simulink model "REF"  (R2025b)
settings: Solver=VariableStepAuto  StartTime=0.0  StopTime=70  RelTol=1e-3
values from neighbouring files (symbols this model uses):
  A_pos_speed = [ zeros(3,3),  eye(3) ... (first row only)    [ref.m]
  Ac_roll = [1]    [ref.m]
  Ac_thrust = [0.92]    [ref.m]
  Ac_yaw = [1]    [ref.m]
  Ad_2 = sys_d_2.A    [ref.m]
  B_pos_speed = [zeros(3,3) ... (first row only)    [ref.m]
  b_roll = 0.02    [ref.m]
  Bc_roll = [1/wn_roll^2 2*ksi_roll/wn_roll 1]    [ref.m]
  Bc_thrust = [0.04 1]    [ref.m]
  Bc_yaw = [0.4 1]    [ref.m]
  Bd_2 = sys_d_2.B    [ref.m]
  C_pos_speed = [eye(6)]    [ref.m]
  D_pos_speed = [zeros(6,3)]    [ref.m]
  delay = 0.08    [ref.m]
  delay_roll = 0.13    [ref.m]
  ekf_model = c2d(tf(1, [0.01 1]), Ts)    [ref.m]
  g = 9.81    [ref.m]
  GLOBAL_PARAMETERS = [Ts m g]    [ref.m]
  initial_pos_conditions_M1 = [0 0 1]'    [ref.m]
  Ki = K_aug(:,7:9)    [ref.m]
  Kx = K_aug(:,1:6)    [ref.m]
  m = 0.075    [ref.m]
  roll_max = 0.25    [ref.m]
  roll_min = -0.25    [ref.m]
  Tmax = 1.0088    [ref.m]
  Tmin = 0.4786    [ref.m]
  Ts = 0.01    [ref.m]
undefined symbols (not defined in the file or in its folder): DiscIntNeverNeededParam
libraries: simulink x2
settings Model: Creator=susbielp  LastModifiedBy=dharani
settings DebuggingCC: UnconnectedInputMsg=warning  UnconnectedOutputMsg=warning  UnconnectedLineMsg=warning
settings ModelReferenceCC: EnableRefExpFcnMdlSchedulingChecks=on
settings RTWCC: GPUComputeCapability=3.5  DLArmComputeVersion=19.05
settings SimscapeCC: SimscapeLogDataHistory=5000  SimscapeLogDecimation=1

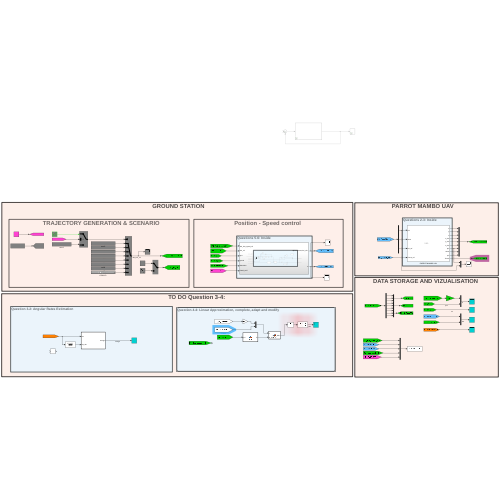
[thumbnail: Simulink's stored preview of the top-level diagram]
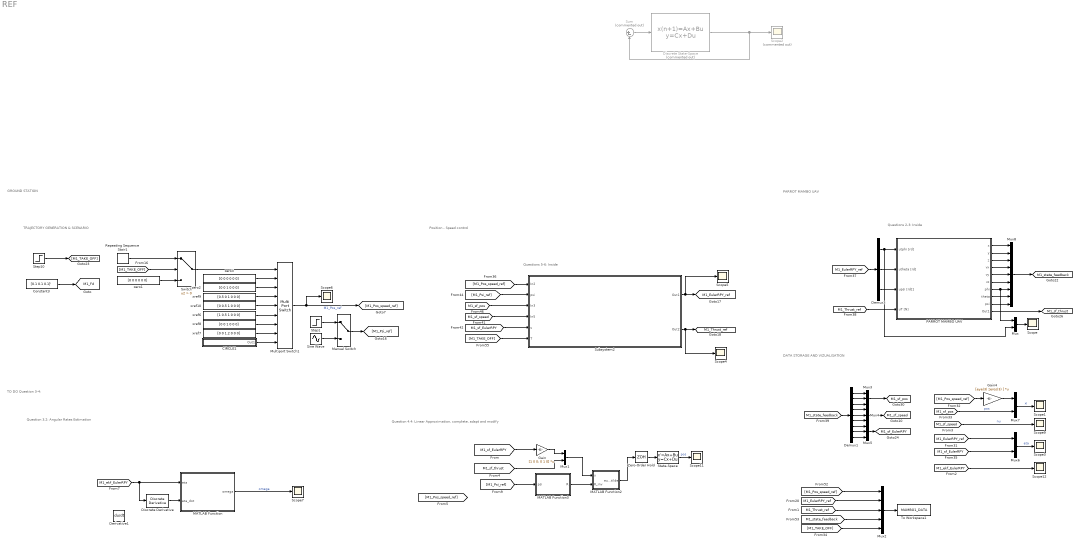
== system REF ==
  note: PARROT MAMBO UAV
  note: TRAJECTORY GENERATION & SCENARIO
  note: DATA STORAGE AND VIZUALISATION
  note: Position - Speed control
  note: GROUND STATION
  note: TO DO Question 3-4:
  note: Question 3.2: Angular Rates Estimation
  note: Question 4.4: Linear Approximation, complete, adapt and modify
  note: Questions 2-3: Inside
  note: Questions 5-6: Inside
  CIRCLE1 : Subsystem
  Constant3 : Constant  Value=[0.1 0.1 0.1]'
  Demux1 : Demux  Outputs=9
  Demux3 : Demux  Outputs=3
  Derivative1 : Derivative
  Discrete Derivative : simulink/Discrete/Discrete Derivative  gainval=1.0  ICPrevScaledInput=0.0  OutMin=[]  OutMax=[]  OutDataType=fixdt(1, 16)  OutScaling=2^-10  DoSatur=off
  Discrete State-Space : DiscreteStateSpace  Commented=on  A=Ad_2  B=Bd_2  C=eye(6)  D=zeros(6,3)  SampleTime=-1
  Gain : Gain  Gain=[1 0 0; 0 1 0]  Multiplication=Matrix(K*u)
  Gain4 : Gain  Gain=[eye(3) zeros(3) ]  Multiplication=Matrix(K*u) (u vector)
  MATLAB Function : MATLAB Function  TreatAsAtomicUnit=on
  MATLAB Function2 : MATLAB Function  TreatAsAtomicUnit=on
  MATLAB Function3 : MATLAB Function  TreatAsAtomicUnit=on
  Manual Switch : ManualSwitch
  Multiport Switch1 : MultiPortSwitch  DataPortOrder=Zero-based contiguous  Inputs=8  zeroidx=on  SaturateOnIntegerOverflow=off  InputSameDT=off
  Mux{,1,6..7} (4 alike) : Mux  Inputs=2
  Mux2 : Mux  Inputs=5
  Mux3 : Mux  Inputs=3
  Mux4 : Mux  Inputs=3
  Mux5 : Mux  Inputs=3
  Mux8 : Mux  Inputs=9
  PARROT MAMBO UAV : Subsystem
      mask Display: image('MAMBO.jpg');
  Repeating Sequence Stair1 : simulink/Sources/Repeating Sequence Stair  OutValues=[1 2 1 3 1 4 1].'  tsamp=10  OutMin=[]  OutMax=[]  OutDataTypeStr=double  OutputDataTypeScalingMode=double  OutDataType=fixdt(0,8)  ConRadixGroup=Best Precision: Vector-wise  OutScaling=2^-12
  Scope{,1,3..7,9,11..12} (10 alike) : Scope
      Scope settings: ActiveDisplayYMinimum=-4718.6931607631386  ActiveDisplayYMaximum=42468.438446868255
      Scope1 settings: ActiveDisplayYMinimum=-0.22929503999038037  ActiveDisplayYMaximum=1.1424783933788982
      Scope11 settings: ActiveDisplayYMinimum=-1.2264719660775174E+8  ActiveDisplayYMaximum=1.1038232126175931E+9
      Scope12 settings: ActiveDisplayYMinimum=-1  ActiveDisplayYMaximum=1  DataLoggingVariableName=ScopeData3
      Scope3 settings: ActiveDisplayYMinimum=-4.6224364909389761  ActiveDisplayYMaximum=4.7084688655508389  DataLoggingVariableName=ScopeData2
      Scope4 settings: ActiveDisplayYMinimum=0.34636950171863107  ActiveDisplayYMaximum=3.6151004918254133  DataLoggingVariableName=ScopeData9
      Scope5 settings: ActiveDisplayYMinimum=-3.4681762236688183  ActiveDisplayYMaximum=6.078387539812379  DataLoggingVariableName=ScopeData10
      Scope6 settings: ActiveDisplayYMinimum=-1  ActiveDisplayYMaximum=1  DataLoggingVariableName=ScopeData4
      Scope7 settings: ActiveDisplayYMinimum=-2.2056944622868526  ActiveDisplayYMaximum=2.1202611493653283  DataLoggingVariableName=ScopeData2
      Scope9 settings: ActiveDisplayYMinimum=-2.6898356842666646  ActiveDisplayYMaximum=2.4869610141324947  DataLoggingVariableName=ScopeData3
  Scope2 : Scope  Commented=on
      settings: DataLoggingVariableName=ScopeData8
  Sine Wave : Sin  SampleTime=0
  State-Space : StateSpace  A=A_pos_speed  B=B_pos_speed  C=C_pos_speed  D=D_pos_speed  InitialCondition=0
  Step1 : Step  Time=25  After=0  SampleTime=0
  Step10 : Step  Time=2  SampleTime=0
  Subsystem2 : Subsystem
  Sum : Sum  Commented=on  Inputs=|+-
  Switch : Switch  Criteria=u2 > Threshold  SaturateOnIntegerOverflow=off  InputSameDT=off
  To Workspace1 : ToWorkspace  VariableName=MAMBO1_DATA  SaveFormat=Timeseries  SampleTime=-1
  Zero-Order Hold : ZeroOrderHold  SampleTime=Ts
  xref10 : Constant  Value=[0 0.5 1 0 0 0]  OutDataTypeStr=double
  xref6 : Constant  Value=[1 0.5 1 0 0 0]  OutDataTypeStr=double
  xref7 : Constant  Value=[0 0 1.2 0 0 0]  OutDataTypeStr=double
  xref8 : Constant  Value=[0 0 1 0 0 0]  OutDataTypeStr=double
  xref9 : Constant  Value=[0.5 0 1 0 0 0]  OutDataTypeStr=double
  zero1 : Constant  Value=[0 0 0 0 0 0]  OutDataTypeStr=double
  zero2 : Constant  Value=[0 0 1 0 0 0]  OutDataTypeStr=double
  zero3 : Constant  Value=[0 0 0 0 0 0]  OutDataTypeStr=double
  tag scope: M1_EulerRPY_ref=global, M1_Fd=global, M1_Thrust_ref=global, M1_sf_EulerRPY=global, M1_sf_pos=global, M1_sf_speed=global, M1_sf_thrust=global, M1_state_feedback=global
  wires:
  Demux3/1 -> Mux/2, PARROT MAMBO UAV/1(utphi [rd])
  Mux5/1 -> [M1_sf_EulerRPY]
  Demux1/4 -> Mux4/1
  [M1_Psi_ref] -> Subsystem2/2(psi)
  PARROT MAMBO UAV/6(vz) -> Mux8/6
  Mux2/1 -> To Workspace1/1
  Demux1/1 -> Mux3/1
  Demux1/3 -> Mux3/3
  Demux3/2 -> PARROT MAMBO UAV/2(utheta [rd])
  Demux3/3 -> PARROT MAMBO UAV/3(upsi [rd]1)
  [M1_sf_pos] -> Mux7/2  "pos"
  Mux7/1 -> Scope1/1  "xi"
  Demux1/6 -> Mux4/3
  PARROT MAMBO UAV/2(y) -> Mux8/2
  PARROT MAMBO UAV/5(vy) -> Mux8/5
  PARROT MAMBO UAV/3(z) -> Mux8/3
  Demux1/5 -> Mux4/2
  [M1_sf_EulerRPY] -> Subsystem2/5(u)
  PARROT MAMBO UAV/9(psi) -> Mux8/9
  Demux1/7 -> Mux5/1
  [M1_sf_EulerRPY] -> Mux6/2
  [M1_sf_speed] -> Subsystem2/4(In5)
  PARROT MAMBO UAV/1(x) -> Mux8/1
  [M1_Pos_speed_ref] -> Subsystem2/1(In2)
  Demux1/2 -> Mux3/2
  PARROT MAMBO UAV/10(Out1) -> [M1_sf_thrust]
  Demux1/8 -> Mux5/2
  Mux4/1 -> [M1_sf_speed]
  [M1_sf_pos] -> Subsystem2/3(In3)
  [M1_EulerRPY_ref] -> Mux6/1
  Mux6/1 -> Scope3/1  "eta"
  [M1_EulerRPY_ref] -> Demux3/1
  Gain4/1 -> Mux7/1
  PARROT MAMBO UAV/8(theta) -> Mux8/8
  PARROT MAMBO UAV/4(vx) -> Mux8/4
  [M1_Pos_speed_ref] -> Gain4/1
  [M1_TAKE_OFF] -> Mux2/5
  [M1_TAKE_OFF] -> Subsystem2/6(T)
  [M1_Thrust_ref] -> PARROT MAMBO UAV/4(uT [N])
  Mux8/1 -> [M1_state_feedback]
  PARROT MAMBO UAV/7(phi) -> Mux/1, Mux8/7
  [M1_EulerRPY_ref] -> Mux2/2
  [M1_state_feedback] -> Demux1/1
  [M1_state_feedback] -> Mux2/4
  Subsystem2/2(Out2) -> Scope4/1, [M1_Thrust_ref]
  Mux3/1 -> [M1_sf_pos]
  Subsystem2/1(Out1) -> Scope5/1, [M1_EulerRPY_ref]
  Demux1/9 -> Mux5/3
  [M1_Pos_speed_ref] -> Mux2/1
  Step10/1 -> [M1_TAKE_OFF]
  CIRCLE1/1(Out1) -> Multiport Switch1/9
  zero3/1 -> Multiport Switch1/2
  Multiport Switch1/1 -> Scope6/1, [M1_Pos_speed_ref]  "M1_Pos_ref"
  xref8/1 -> Multiport Switch1/7
  xref7/1 -> Multiport Switch1/8
  xref9/1 -> Multiport Switch1/4
  xref10/1 -> Multiport Switch1/5
  zero2/1 -> Multiport Switch1/3
  xref6/1 -> Multiport Switch1/6
  [M1_Thrust_ref] -> Mux2/3
  Manual Switch/1 -> [M1_Psi_ref]
  Switch/1 -> Multiport Switch1/1
  [M1_TAKE_OFF] -> Switch/2
  zero1/1 -> Switch/3
  Repeating Sequence Stair1/1 -> Switch/1
  State-Space/1 -> Scope11/1  "pos"
  Step1/1 -> Manual Switch/1
  Sine Wave/1 -> Manual Switch/2
  [M1_sf_speed] -> Scope9/1  "nu"
  [M1_ekf_EulerRPY] -> Scope12/1
  Zero-Order Hold/1 -> State-Space/1
  Constant3/1 -> [M1_Fd]
  [M1_ekf_EulerRPY] -> MATLAB Function/1(eta), Discrete Derivative/1
  Mux/1 -> Scope/1
  MATLAB Function/1(omega) -> Scope7/1  "omega"
  [M1_sf_EulerRPY] -> Gain/1
  Mux1/1 -> MATLAB Function2/1(u)
  Gain/1 -> Mux1/1
  [M1_sf_thrust] -> Mux1/2
  MATLAB Function3/1(R) -> MATLAB Function2/2(R_inv)
  [M1_Psi_ref] -> MATLAB Function3/1(psi)
  MATLAB Function2/1(euler_tilde) -> Zero-Order Hold/1
  Discrete State-Space/1 -> Sum/2, Scope2/1
  Sum/1 -> Discrete State-Space/1
  Discrete Derivative/1 -> MATLAB Function/2(eta_dot)

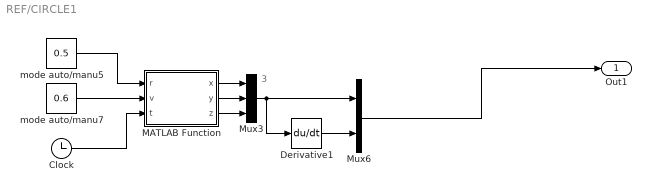
== system REF/CIRCLE1 ==
  note: 3
  Clock : Clock
  Derivative1 : Derivative  CoefficientInTFapproximation=4*Ts
  MATLAB Function : MATLAB Function  TreatAsAtomicUnit=on
  Mux3 : Mux  Inputs=3
  Mux6 : Mux  Inputs=2
  mode auto/manu5 : Constant  Value=0.5  OutDataTypeStr=double
  mode auto/manu7 : Constant  Value=0.6  OutDataTypeStr=double
  Out1 : Outport
  wires:
  MATLAB Function/2(y) -> Mux3/2
  Derivative1/1 -> Mux6/2
  Mux3/1 -> Mux6/1, Derivative1/1
  Mux6/1 -> Out1/1
  mode auto/manu5/1 -> MATLAB Function/1(r)
  Clock/1 -> MATLAB Function/3(t)
  MATLAB Function/1(x) -> Mux3/1
  mode auto/manu7/1 -> MATLAB Function/2(v)
  MATLAB Function/3(z) -> Mux3/3

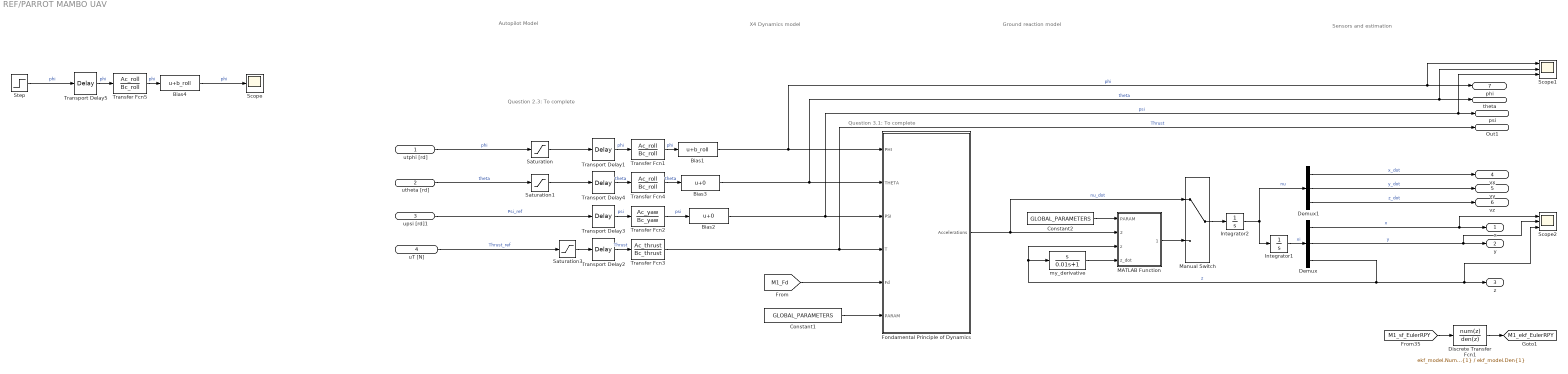
== system REF/PARROT MAMBO UAV ==
  note: Sensors and estimation
  note: X4 Dynamics model
  note: Ground reaction model
  note: Autopilot Model
  note: Question 2.3: To complete
  note: Question 3.1: To complete
  utphi [rd] : Inport
  utheta [rd] : Inport  Port=2
  upsi [rd]1 : Inport  Port=3
  uT [N] : Inport  Port=4
  Bias1 : Bias  Bias=b_roll  SaturateOnIntegerOverflow=off
  Bias2 : Bias  SaturateOnIntegerOverflow=off
  Bias3 : Bias  SaturateOnIntegerOverflow=off
  Bias4 : Bias  Bias=b_roll  SaturateOnIntegerOverflow=off
  Constant1 : Constant  Value=GLOBAL_PARAMETERS
  Constant2 : Constant  Value=GLOBAL_PARAMETERS
  Demux : Demux  Outputs=3
  Demux1 : Demux  Outputs=3
  Discrete Transfer Fcn1 : DiscreteTransferFcn  Numerator=ekf_model.Num{1}  Denominator=ekf_model.Den{1}  SampleTime=Ts
  Fondamental Principle of Dynamics : MATLAB Function  TreatAsAtomicUnit=on
  Integrator1 : Integrator  InitialCondition=initial_pos_conditions_M1
  Integrator2 : Integrator  InitialCondition=[0 0 0]'
  MATLAB Function : MATLAB Function  TreatAsAtomicUnit=on
  Manual Switch : ManualSwitch
  Saturation : Saturate  UpperLimit=roll_max  LowerLimit=roll_min
  Saturation1 : Saturate  UpperLimit=roll_max  LowerLimit=roll_min
  Saturation3 : Saturate  UpperLimit=Tmax  LowerLimit=Tmin
  Scope : Scope
      settings: ActiveDisplayYMinimum=-1  ActiveDisplayYMaximum=1  DataLoggingVariableName=ScopeData5
  Scope1 : Scope  NumInputPorts=3
      settings: ActiveDisplayYMinimum=-1  ActiveDisplayYMaximum=1  DataLoggingVariableName=ScopeData6
  Scope2 : Scope  NumInputPorts=3
      settings: ActiveDisplayYMinimum=-11359.713997262726  ActiveDisplayYMaximum=2011.2230868177148  DataLoggingVariableName=ScopeData7
  Step : Step  SampleTime=0
  Transfer Fcn1 : TransferFcn  Numerator=Ac_roll  Denominator=Bc_roll
  Transfer Fcn2 : TransferFcn  Numerator=Ac_yaw  Denominator=Bc_yaw
  Transfer Fcn3 : TransferFcn  Numerator=Ac_thrust  Denominator=Bc_thrust
  Transfer Fcn4 : TransferFcn  Numerator=Ac_roll  Denominator=Bc_roll
  Transfer Fcn5 : TransferFcn  Numerator=Ac_roll  Denominator=Bc_roll
  Transport Delay1 : TransportDelay  DelayTime=delay_roll
  Transport Delay2 : TransportDelay  DelayTime=delay
  Transport Delay3 : TransportDelay  DelayTime=delay
  Transport Delay4 : TransportDelay  DelayTime=delay_roll
  Transport Delay5 : TransportDelay  DelayTime=delay_roll
  my_derivative : TransferFcn  Numerator=[1 0]  Denominator=[0.01 1]
  x : Outport  VectorParamsAs1DForOutWhenUnconnected=off
  y : Outport  Port=2  VectorParamsAs1DForOutWhenUnconnected=off
  z : Outport  Port=3  VectorParamsAs1DForOutWhenUnconnected=off
  vx : Outport  Port=4  VectorParamsAs1DForOutWhenUnconnected=off
  vy : Outport  Port=5  VectorParamsAs1DForOutWhenUnconnected=off
  vz : Outport  Port=6  VectorParamsAs1DForOutWhenUnconnected=off
  phi : Outport  Port=7  VectorParamsAs1DForOutWhenUnconnected=off
  theta : Outport  Port=8  VectorParamsAs1DForOutWhenUnconnected=off
  psi : Outport  Port=9  VectorParamsAs1DForOutWhenUnconnected=off
  Out1 : Outport  Port=10
  tag scope: M1_ekf_EulerRPY=global
  wires:
  uT [N]/1 -> Saturation3/1  "Thrust_ref"
  Integrator2/1 -> Integrator1/1, Demux1/1  "nu"
  Demux1/1 -> vx/1  "x_dot"
  Saturation3/1 -> Transport Delay2/1
  Fondamental Principle of Dynamics/1(Accelerations) -> Manual Switch/1, MATLAB Function/2(Accelerations_model)  "nu_dot"
  Transport Delay2/1 -> Transfer Fcn3/1  "Thrust"
  Demux1/3 -> vz/1  "z_dot"
  upsi [rd]1/1 -> Transport Delay3/1  "Psi_ref"
  Constant1/1 -> Fondamental Principle of Dynamics/6(PARAM)
  Demux1/2 -> vy/1  "y_dot"
  Integrator1/1 -> Demux/1  "xi"
  Transport Delay3/1 -> Transfer Fcn2/1  "psi"
  Demux/1 -> Scope2/1, x/1  "x"
  Demux/2 -> Scope2/2, y/1  "y"
  Transfer Fcn3/1 -> Fondamental Principle of Dynamics/4(T), Out1/1  "Thrust"
  Demux/3 -> my_derivative/1, MATLAB Function/3(z), Scope2/3, z/1  "z"
  Transfer Fcn2/1 -> Bias2/1  "psi"
  Bias2/1 -> Fondamental Principle of Dynamics/3(PSI), Scope1/3, psi/1  "psi"
  my_derivative/1 -> MATLAB Function/4(z_dot)
  MATLAB Function/1(Accelerations) -> Manual Switch/2
  [M1_Fd] -> Fondamental Principle of Dynamics/5(Fd)
  Constant2/1 -> MATLAB Function/1(PARAM)
  Discrete Transfer Fcn1/1 -> [M1_ekf_EulerRPY]
  [M1_sf_EulerRPY] -> Discrete Transfer Fcn1/1
  Manual Switch/1 -> Integrator2/1
  Transport Delay4/1 -> Transfer Fcn4/1  "theta"
  Transfer Fcn4/1 -> Bias3/1  "theta"
  Bias3/1 -> Scope1/2, theta/1, Fondamental Principle of Dynamics/2(THETA)  "theta"
  Transport Delay1/1 -> Transfer Fcn1/1  "phi"
  Transfer Fcn1/1 -> Bias1/1  "phi"
  Bias1/1 -> Scope1/1, phi/1, Fondamental Principle of Dynamics/1(PHI)  "phi"
  Step/1 -> Transport Delay5/1  "phi"
  Bias4/1 -> Scope/1  "phi"
  Transfer Fcn5/1 -> Bias4/1  "phi"
  Transport Delay5/1 -> Transfer Fcn5/1  "phi"
  Saturation/1 -> Transport Delay1/1
  utphi [rd]/1 -> Saturation/1  "phi"
  Saturation1/1 -> Transport Delay4/1
  utheta [rd]/1 -> Saturation1/1  "theta"

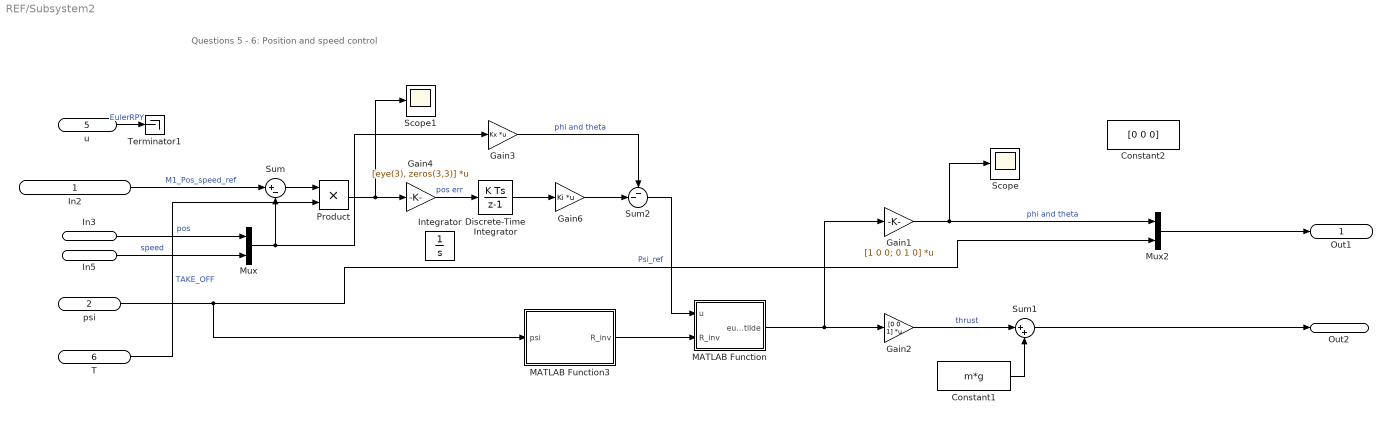
== system REF/Subsystem2 ==
  note: Questions 5 - 6: Position and speed control
  In2 : Inport
  psi : Inport  Port=2
  In3 : Inport  Port=3
  In5 : Inport  Port=4
  u : Inport  Port=5
  T : Inport  Port=6
  Constant1 : Constant  Value=m*g
  Constant2 : Constant  Value=[0 0 0]
  Discrete-Time Integrator : DiscreteIntegrator  SampleTime=-1  ICPrevOutput=DiscIntNeverNeededParam  ICPrevScaledInput=DiscIntNeverNeededParam
  Gain1 : Gain  Gain=[1 0 0; 0 1 0]  Multiplication=Matrix(K*u)
  Gain2 : Gain  Gain=[0 0 1]  Multiplication=Matrix(K*u)
  Gain3 : Gain  Gain=Kx  Multiplication=Matrix(K*u)
  Gain4 : Gain  Gain=[eye(3), zeros(3,3)]  Multiplication=Matrix(K*u)
  Gain6 : Gain  Gain=Ki  Multiplication=Matrix(K*u)
  Integrator : Integrator
  MATLAB Function : MATLAB Function  TreatAsAtomicUnit=on
  MATLAB Function3 : MATLAB Function  TreatAsAtomicUnit=on
  Mux : Mux  Inputs=2
  Mux2 : Mux  Inputs=2
  Product : Product
  Scope : Scope
      settings: ActiveDisplayYMinimum=-1  ActiveDisplayYMaximum=1  DataLoggingVariableName=ScopeData11
  Scope1 : Scope
      settings: ActiveDisplayYMinimum=-143.0702716601204  ActiveDisplayYMaximum=95.933051940311913  DataLoggingVariableName=ScopeData12
  Sum : Sum  Inputs=|+-
  Sum1 : Sum  Inputs=|++
  Sum2 : Sum  Inputs=--|
  Terminator1 : Terminator
  Out1 : Outport
  Out2 : Outport  Port=2
  wires:
  Mux2/1 -> Out1/1
  In2/1 -> Sum/1  "M1_Pos_speed_ref"
  In3/1 -> Mux/1  "pos"
  In5/1 -> Mux/2  "speed"
  psi/1 -> MATLAB Function3/1(psi), Mux2/2  "Psi_ref"
  MATLAB Function3/1(R_inv) -> MATLAB Function/2(R_inv)
  Gain1/1 -> Scope/1, Mux2/1  "phi and theta"
  MATLAB Function/1(euler_tilde) -> Gain2/1, Gain1/1
  Gain2/1 -> Sum1/1  "thrust"
  Sum1/1 -> Out2/1
  Constant1/1 -> Sum1/2
  Mux/1 -> Gain3/1, Sum/2
  T/1 -> Product/2  "TAKE_OFF"
  u/1 -> Terminator1/1  "EulerRPY"
  Sum2/1 -> MATLAB Function/1(u)
  Gain6/1 -> Sum2/2
  Gain3/1 -> Sum2/1  "phi and theta"
  Gain4/1 -> Discrete-Time Integrator/1  "pos err"
  Discrete-Time Integrator/1 -> Gain6/1
  Sum/1 -> Product/1
  Product/1 -> Scope1/1, Gain4/1

== matlab function REF/MATLAB Function ==
  data: omega output; eta input; eta_dot input
function omega =  compute_omega(eta,eta_dot)
    phi= eta(1);
    theta = eta(2);
    psi = eta(3);
    inv_T = [1     0       -sin(theta);
             0 cos(phi) sin(phi)*cos(theta);
             0 -sin(phi) cos(phi)*cos(theta)];
omega = inv_T*eta_dot;

== matlab function REF/PARROT MAMBO UAV/MATLAB Function ==
  data: PARAM input; Accelerations_model input; Accelerations output; z input; z_dot input
function Accelerations = ground_model(PARAM, Accelerations_model, z, z_dot)

    Ts = PARAM(1) ;
    m = PARAM(2) ;
    g = PARAM(3) ; 

    Accelerations = Accelerations_model ; 
    if z < 0.01 
        Accelerations =  [0 0 Accelerations_model(3)]' + [0 0 -m*g*100*(z - 0.01)]' - [0 0 10*z_dot]' ;
    end
    if Accelerations_model == [0 0 0]'  
        Accelerations = [0 0 0]';
    end
end

== matlab function REF/CIRCLE1/MATLAB Function ==
  data: x output; r input; y output; v input; t input; z output
function [x,y,z]= fcn(r,v,t)
w=v/r;
x=r*cos(w*t);
y=r*sin(w*t);
z=1;

== matlab function REF/MATLAB Function2 ==
  data: u input; euler_tilde output; R_inv input
function euler_tilde = fcn(u,R_inv)

euler_tilde = R_inv*u;

== matlab function REF/Subsystem2/MATLAB Function ==
  data: u input; euler_tilde output; R_inv input
function euler_tilde = fcn(u,R_inv)

euler_tilde = R_inv*u;

== matlab function REF/Subsystem2/MATLAB Function3 ==
  data: psi input; R_inv output
function  R_inv = fcn(psi)
    % Change of variable
    R_inv = [ cos(psi) -sin(psi) 0;
          sin(psi) cos(psi) 0;
          0 0 1]';

== matlab function REF/MATLAB Function3 ==
  data: psi input; R output
function  R = fcn(psi)
    % Change of variable
    R = [ cos(psi) -sin(psi) 0;
          sin(psi) cos(psi) 0;
          0 0 1];

== matlab function REF/PARROT MAMBO UAV/Fondamental Principle of Dynamics ==
  data: PHI input; Accelerations output; THETA input; PSI input; T input; Fd input; PARAM input
function Accelerations = fcn(PHI, THETA, PSI, T, Fd, PARAM)
    m = PARAM(2);
    g = PARAM(3);
    
    % Rotation matrix R(φ, θ, ψ)
    cphi = cos(PHI);   sphi = sin(PHI);
    ctheta = cos(THETA); stheta = sin(THETA);
    cpsi = cos(PSI);   spsi = sin(PSI);
    
    R = [cpsi*ctheta, cpsi*stheta*sphi - spsi*cphi, cpsi*stheta*cphi + spsi*sphi;
         spsi*ctheta, spsi*stheta*sphi + cpsi*cphi, spsi*stheta*cphi - cpsi*sphi;
         -stheta,     ctheta*sphi,                  ctheta*cphi];
    
    % Acceleration: mν̇ = -mg*e3 + R'*T + Fd
    % ν̇ = (-mg*e3 + R'*[0; 0; T] + Fd) / m
    Thrust_vector = [0; 0; T];
    gravity_vector = [0; 0; -m*g];
    
    Accelerations = (gravity_vector + R * Thrust_vector + Fd) / m;
end
